simulink library "RLAgent"  (R2026a)
settings: Solver=VariableStepAuto
settings Model: Creator=abhinav  LastModifiedBy=abhinav

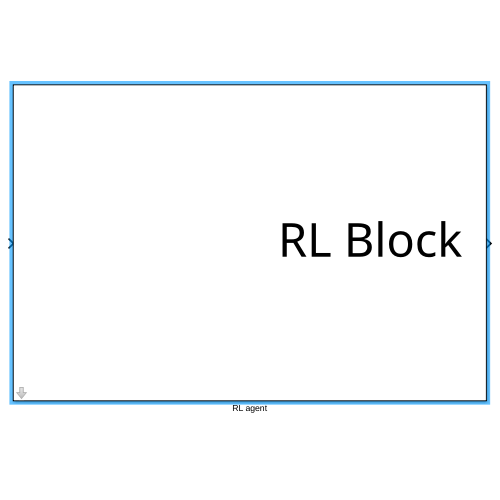
[thumbnail: Simulink's stored preview of the top-level diagram]
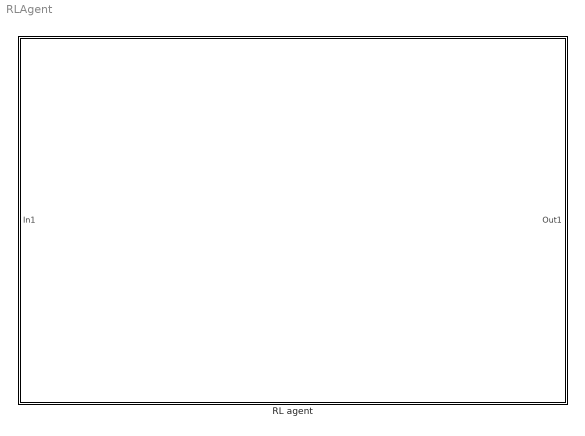
== system RLAgent ==
  RL agent : Subsystem  mask{Parameter1=0}

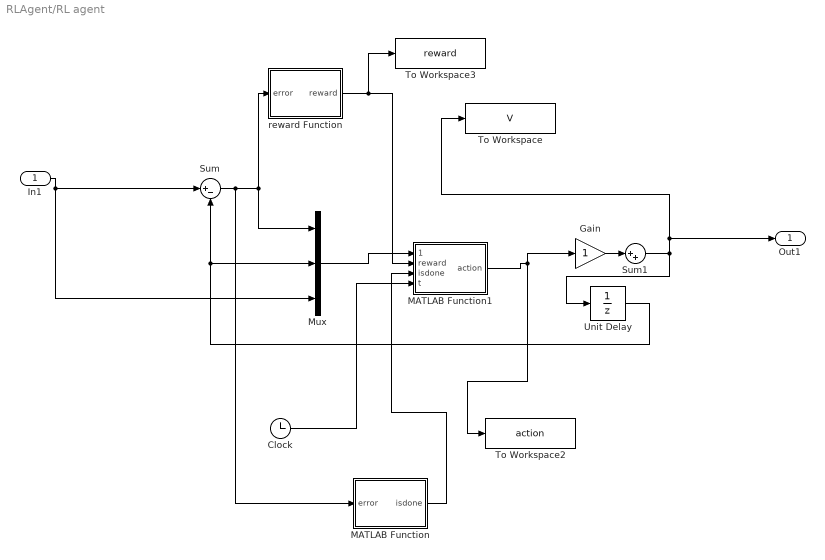
== system RLAgent/RL agent ==
  In1 : Inport
  Clock : Clock
  Gain : Gain
  MATLAB Function : MATLAB Function  TreatAsAtomicUnit=on
  MATLAB Function1 : MATLAB Function  TreatAsAtomicUnit=on
  Mux : Mux  Inputs=3
  Sum : Sum  Inputs=|+-
  Sum1 : Sum  Inputs=|++
  To Workspace : ToWorkspace  VariableName=V  SampleTime=-1
  To Workspace2 : ToWorkspace  VariableName=action  SampleTime=-1
  To Workspace3 : ToWorkspace  VariableName=reward  SaveFormat=Timeseries  SampleTime=-1
  Unit Delay : UnitDelay
  reward Function : MATLAB Function  TreatAsAtomicUnit=on
  Out1 : Outport
  wires:
  Clock/1 -> MATLAB Function1/4(t)
  Gain/1 -> Sum1/1
  MATLAB Function/1(isdone) -> MATLAB Function1/3(isdone)
  In1/1 -> Sum/1, Mux/3
  reward Function/1(reward) -> MATLAB Function1/2(reward), To Workspace3/1
  Mux/1 -> MATLAB Function1/1(observation)
  Unit Delay/1 -> Mux/2, Sum/2
  MATLAB Function1/1(action) -> To Workspace2/1, Gain/1
  Sum1/1 -> Out1/1, To Workspace/1, Unit Delay/1
  Sum/1 -> MATLAB Function/1(error), Mux/1, reward Function/1(error)

== matlab function RLAgent/RL agent/MATLAB Function ==
  data: error input; isdone output
function isdone = fcn(error)
isdone = abs(error) > 350;
end
%#codegen

== matlab function RLAgent/RL agent/reward Function ==
  data: error input; reward output

%#codegen
function reward = fcn(error)
    reward = -error^2;
end

== matlab function RLAgent/RL agent/MATLAB Function1 ==
  data: observation input; action output; reward input; isdone input; t input
function action = fcn(observation, reward, isdone, t)
persistent W b bestW bestb bestReward totalReward episodeStartTime

if isempty(W)
    W = 0.01 * randn(1,3);
    b = 150;
    bestW = W; bestb = b;
    bestReward = -Inf;
    totalReward = 0;
    episodeStartTime = 0;
end

obsNorm = observation / 300;
action = W * obsNorm + b;
action = min(max(action, 0), 350);

totalReward = totalReward + reward;

episodeLength = 10;   % seconds per "episode"
episodeEnd = (t - episodeStartTime) >= episodeLength;

if episodeEnd
    if totalReward > bestReward
        bestReward = totalReward;
        bestW = W;
        bestb = b;
    else
        W = bestW;
        b = bestb;
    end

    W = bestW + 0.5*randn(size(bestW));
    b = bestb + 5*randn;

    totalReward = 0;
    episodeStartTime = t;
end
end
